simulink model "modele_freinage_regeneratif_v1"  (R2024a)
settings: Solver=VariableStepAuto  StartTime=0.0  StopTime=10.0  RelTol=1e-3
settings Model: Creator=HP  LastModifiedBy=HP

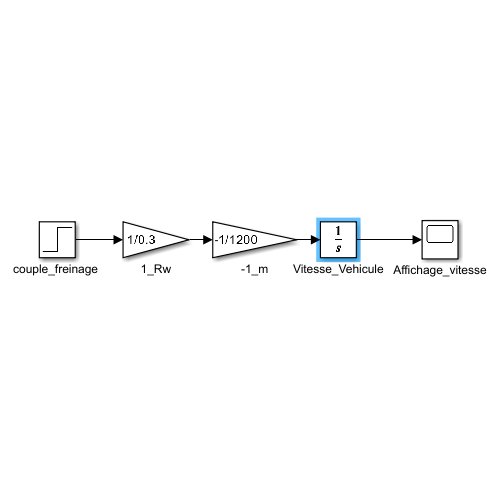
[thumbnail: Simulink's stored preview of the top-level diagram]
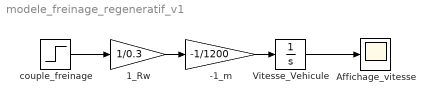
== system modele_freinage_regeneratif_v1 ==
  -1_m : Gain  Gain=-1/1200
  1_Rw : Gain  Gain=1/0.3
  Affichage_vitesse : Scope
  Vitesse_Vehicule : Integrator  InitialCondition=20
  "couple_freinage " : Step  After=150  SampleTime=0
  wires:
  "couple_freinage "/1 -> 1_Rw/1
  1_Rw/1 -> -1_m/1
  -1_m/1 -> Vitesse_Vehicule/1
  Vitesse_Vehicule/1 -> Affichage_vitesse/1
